simulink model "blance_leg2_machined"  (R2023a)
settings: Solver=VariableStepAuto  StartTime=0.0  StopTime=10  MaxStep=0.0050000000000000001  RelTol=5.0000000000000002e-05  AbsTol=9.9999999999999995e-07
InitFcn:
  | addpath(fileparts(get_param(bdroot,'FileName')));
  | apply_config(bdroot);
model workspace (MAT data in the model file):
  L_length_ref = timeseries
  L_length_ref.Name = 'unnamed'
  L_length_ref.DataInfo = tsdata.datametadata
  L_length_ref.DataInfo.Interpolation = tsdata.interpolation
  L_length_ref.DataInfo.Interpolation.Fhandle : function handle (value not decoded)
  L_length_ref.DataInfo.Interpolation.Name = 'linear'
  L_length_ref.TimeInfo = tsdata.timemetadata
  L_length_ref.TimeInfo.Length = 2
  L_length_ref.TimeInfo.DuplicateTimes = 0
  L_length_ref.TimeInfo.Time_ = [0; 10]
  L_length_ref.TimeInfo.Initialized = 1
  L_length_ref.QualityInfo = tsdata.qualmetadata
  L_length_ref.Data_ = [0.08; 0.08]
  L_v_ref = timeseries
  L_v_ref.Name = 'unnamed'
  L_v_ref.DataInfo = tsdata.datametadata
  L_v_ref.DataInfo.Interpolation = tsdata.interpolation
  L_v_ref.DataInfo.Interpolation.Fhandle : function handle (value not decoded)
  L_v_ref.DataInfo.Interpolation.Name = 'linear'
  L_v_ref.TimeInfo = tsdata.timemetadata
  L_v_ref.TimeInfo.Length = 3
  L_v_ref.TimeInfo.DuplicateTimes = 0
  L_v_ref.TimeInfo.Time_ = [0; 2; 5]
  L_v_ref.TimeInfo.Initialized = 1
  L_v_ref.QualityInfo = tsdata.qualmetadata
  L_v_ref.Data_ = [0; 2; 0]
  R_length_ref = timeseries
  R_length_ref.Name = 'unnamed'
  R_length_ref.DataInfo = tsdata.datametadata
  R_length_ref.DataInfo.Interpolation = tsdata.interpolation
  R_length_ref.DataInfo.Interpolation.Fhandle : function handle (value not decoded)
  R_length_ref.DataInfo.Interpolation.Name = 'linear'
  R_length_ref.TimeInfo = tsdata.timemetadata
  R_length_ref.TimeInfo.Length = 2
  R_length_ref.TimeInfo.DuplicateTimes = 0
  R_length_ref.TimeInfo.Time_ = [0; 10]
  R_length_ref.TimeInfo.Initialized = 1
  R_length_ref.QualityInfo = tsdata.qualmetadata
  R_length_ref.Data_ = [0.08; 0.08]
  R_v_ref = timeseries
  R_v_ref.Name = 'unnamed'
  R_v_ref.DataInfo = tsdata.datametadata
  R_v_ref.DataInfo.Interpolation = tsdata.interpolation
  R_v_ref.DataInfo.Interpolation.Fhandle : function handle (value not decoded)
  R_v_ref.DataInfo.Interpolation.Name = 'linear'
  R_v_ref.TimeInfo = tsdata.timemetadata
  R_v_ref.TimeInfo.Length = 3
  R_v_ref.TimeInfo.DuplicateTimes = 0
  R_v_ref.TimeInfo.Time_ = [0; 2; 5]
  R_v_ref.TimeInfo.Initialized = 1
  R_v_ref.QualityInfo = tsdata.qualmetadata
  R_v_ref.Data_ = [0; 2; 0]
  runScenario_cfg_override = []
  wheel_speed_compensation = 1
values from neighbouring files (symbols this model uses):
  K = cachedK    [configured_lqr_gain.m]    (also in get_k_length.m = lqr(A,B,Q,R); matlab.mat = [-1.73670717704  -0.157075032659  -0.691811333866  -0.787613)
  N = NM + mp*diff(x + L*sin(theta),t,2)    [get_k_length.m]
  s = sin(phi3 - phi2)    [five_bar_geometry_rm.m]
undefined symbols (not defined in the file or in its folder): X, Y, Z
libraries: sm_lib x82, nesl_utility x35, slpidlib x2
(part 1 of 3)
settings Model: Creator=Hhop  LastModifiedBy=2024r9000p
settings SolverCC: AlgebraicLoopSolver=TrustRegion  MinimalZcImpactIntegration=on
settings DebuggingCC: ReadBeforeWriteMsg=DisableAll  WriteAfterWriteMsg=DisableAll  WriteAfterReadMsg=DisableAll  MultiTaskDSMMsg=none
settings ModelReferenceCC: UpdateModelReferenceTargets=IfOutOfDate
settings SFSimCC: SFSimEcho=off
settings RTWCC: DLArmComputeVersion=19.05
settings ExplorerConfigSet: InternalSimMechanicsExplorerSettings="<ExplorerConfiguration><canonicalview>default</canonicalview><AnimationSetting><BasePlaybackSpeed>1.0</BasePlaybackSpeed><PlaybackSpeedFactor>1.0</PlaybackSpeedFactor></AnimationSetting><TilePanel><TileInfo><Tiles Columns=\"1\" Count=\"1\" Rows=\"1\"><Column Weight=\"1\"/><Row Weight=\"1\"/><Tile Height=\"1\" Width=\"1\" X=\"0\" Y=\"0\"/></Tiles></TileInfo><SceneInfo><SceneViewer><BGColor><R>0.60000002384185791</R><G>0.60000002384185791</G><B>0.60000002384185791</B></BGColor><Camera><DoPerspective>on</DoPerspective><Position><X>0.799859824006459164</X><Y>3.18443911570358829</Y><Z>0.15361581150017517</Z></Position><Center><X>-0.000140175993540658794</X><Y>3.18443911570358829</Y><Z>0.15361581150017517</Z></Center><Up><X>0</X><Y>0</Y><Z>1</Z></Up><ViewLimDist>1</ViewLimDist><YLim>0.466307658154998583</YLim><XLim>0.83228851713119445</XLim></Camera></SceneViewer></SceneInfo></TilePanel><MechEditorPanel><Cameras><Camera><Id>Camera1</Id><Value><Name>Camera1</Name><NativeCamera><PositionTrackingFeature>blance_leg_model.Rigid_Transform6.F</PositionTrackingFeature><CenterTrackingFeature>blance_leg_model.pitch.B</CenterTrackingFeature><UpVectorTrackingFeature>blance_leg_model.World_Frame1.W</UpVectorTrackingFeature><CenterTrackingOrigin>on</CenterTrackingOrigin><UpVectorTrackingDirection>+Z</UpVectorTrackingDirection></NativeCamera></Value></Camera></Cameras><GfxPanelCameraMap><MapElement CameraMLId=\"Camera1\" GfxPanelIndex=\"0\"/></GfxPanelCameraMap><VideoCreator><PlaybackSpeedRatio>1.0</PlaybackSpeedRatio><FrameRate>30</FrameRate><VideoFormat>Motion JPEG AVI</VideoFormat><FrameSize>auto</FrameSize></VideoCreator></MechEditorPanel></ExplorerConfiguration>"

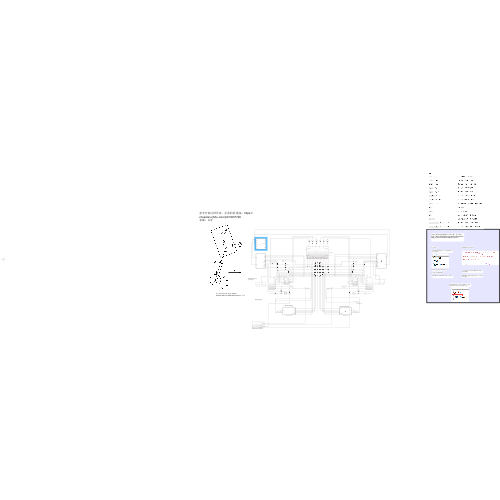
[thumbnail: Simulink's stored preview of the top-level diagram]
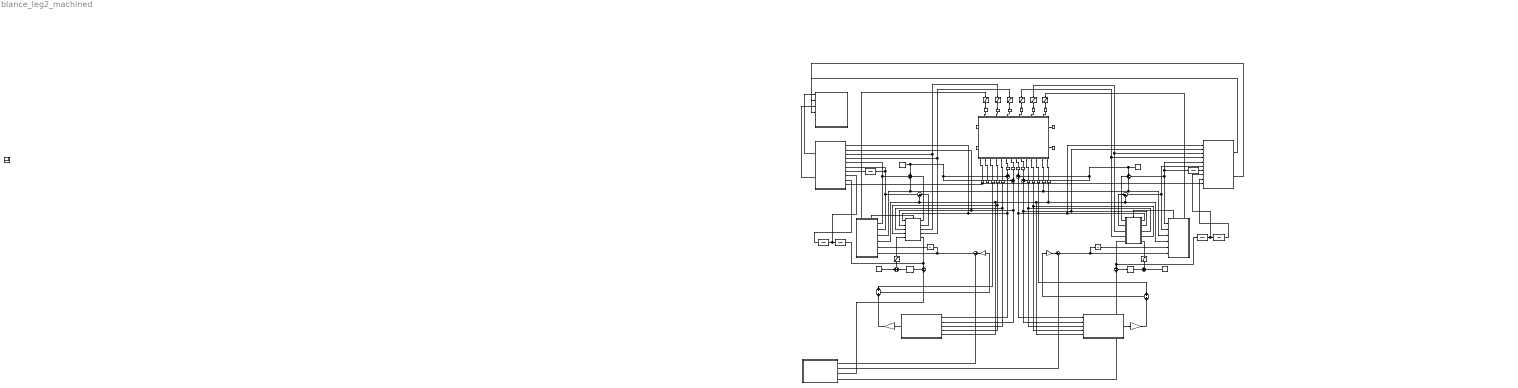
== system blance_leg2_machined ==
  note: 左侧支架对地角速度
  note: 状态目标设置
  note: 二阶系统
  note: LQR输出驱动轮转矩
      | 与虚拟杠转矩
  note: 参考开源文档作者：韭菜的菜 链接：https://zhuanlan.zhihu.com/p/613007726 来源：知乎
  note: 图片来源韭菜的菜 链接：https://zhuanlan.zhihu.com/p/613007726来源：知乎
  note: 运行步骤 :
  note: 所有开源文件必须置于同一文件夹(最好不要使用中文路径)
  note: 得到K参数后进入simulink 点击“运行”开始仿真
  note: addpath'(你所要想添加到的路径)'，具体用法可自行搜索
  note: 如果遇到如下图所示错误
  note: 可点击将其文件夹添加到MATLAB，或输入代码更换路径
  note: K = get_k_length(0.08)
  note: 在命令行窗口运行下图所示代码
  note: 如果想获取K矩阵关于腿长的函数的三次多项式系数在命令行窗口运行下图所示文件
  note: 该仿真是在b站轮腿机器人仿真开源上进行修改，链接：https://www.bilibili.com/read/cv26677904/?spm_id_from=333.999.0.0&jump_opus=1
  note: 右侧支架对地角速度
  Constant10 : Constant  Value=pi/2
  Constant12 : Constant  Value=pi/2
  Gain : Gain  Gain=-0.0603
  Gain1 : Gain  Gain=-0.0603
  Integrator1 : Integrator
  Integrator3 : Integrator
  Left Carrier Compensation Enable : Gain  Gain=wheel_speed_compensation
  Left Ground Wheel Omega : Sum
  Left Wheel Carrier Rate : MATLAB Function  TreatAsAtomicUnit=on
  MATLAB Function : MATLAB Function  TreatAsAtomicUnit=on
  MATLAB Function1 : MATLAB Function  TreatAsAtomicUnit=on
  MATLAB Function2 : MATLAB Function  TreatAsAtomicUnit=on
  PID Controller2 : slpidlib/PID Controller  Controller=PID  Form=Parallel  TimeDomain=Continuous-time  UseExternalTs=off  SampleTime=-1  IntegratorMethod=Forward Euler  FilterMethod=Forward Euler  ControllerParametersSource=internal  P=220  I=0  UseKiTs=off  D=1000  N=100  UseFilter=on  TunerSelectOption=Transfer Function Based (PID Tuner App)  InitialConditionSource=internal  InitialConditionForIntegrator=0  InitialConditionForFilter=0  DifferentiatorICPrevScaledInput=0  ExternalReset=none  TrackingMode=off  Kt=1  LimitOutput=off  SatLimitsSource=internal  UpperSaturationLimit=inf  LowerSaturationLimit=-inf  LinearizeAsGain=on  AntiWindupMode=none  Kb=1  LimitIntegrator=off  UpperIntegratorSaturationLimit=inf  LowerIntegratorSaturationLimit=-inf  POutMin=[]  POutMax=[]  IOutMin=[]  IOutMax=[]  DOutMin=[]  DOutMax=[]  NOutMin=[]  NOutMax=[]  SumOutMin=[]  SumOutMax=[]  SaturationOutMin=[]  SaturationOutMax=[]  PParamMin=[]  PParamMax=[]  IParamMin=[]  IParamMax=[]  DParamMin=[]  DParamMax=[]  NParamMin=[]  NParamMax=[]  KbParamMin=[]  KbParamMax=[]  KtParamMin=[]  KtParamMax=[]  KbOutMin=[]  KbOutMax=[]  KtOutMin=[]  KtOutMax=[]  IntegratorOutMin=[]  IntegratorOutMax=[]  FilterOutMin=[]  FilterOutMax=[]  SumI1OutMin=[]  SumI1OutMax=[]  SumI2OutMin=[]  SumI2OutMax=[]  SumI3OutMin=[]  SumI3OutMax=[]  SumI4OutMin=[]  SumI4OutMax=[]  SumDOutMin=[]  SumDOutMax=[]  DifferentiatorOutMin=[]  DifferentiatorOutMax=[]  FilterDiffOutCoefMin=[]  FilterDiffOutCoefMax=[]  ReciprocalOutMin=[]  ReciprocalOutMax=[]  SumDenOutMin=[]  SumDenOutMax=[]  SumNumOutMin=[]  SumNumOutMax=[]  DivideOutMin=[]  DivideOutMax=[]  UdiffTsProdOutMin=[]  UdiffTsProdOutMax=[]  NTsProdOutMin=[]  NTsProdOutMax=[]  UintegralTsProdOutMin=[]  UintegralTsProdOutMax=[]  UngainTsProdOutMin=[]  UngainTsProdOutMax=[]  ClampingZeroOutDataTypeStr=Inherit: Inherit via back propagation  ClampingZeroOutMin=[]  ClampingZeroOutMax=[]  FilterDenConstantOutDataTypeStr=Inherit: Inherit via back propagation  FilterDenConstantOutMin=[]  FilterDenConstantOutMax=[]  PCopyOutDataTypeStr=Inherit: Inherit via back propagation  PCopyOutMin=[]  PCopyOutMax=[]  NCopyOutDataTypeStr=Inherit: Inherit via back propagation  NCopyOutMin=[]  NCopyOutMax=[]  IntegratorContinuousStateAttributes=''  IntegratorStateMustResolveToSignalObject=off  IntegratorRTWStateStorageClass=Auto  FilterContinuousStateAttributes=''  FilterStateMustResolveToSignalObject=off  FilterRTWStateStorageClass=Auto  ParallelPVariant=InternalParameters  IdealPVariant=Disabled  IVariant=InternalParameters  DVariant=InternalParameters  IntegratorVariant=Continuous  SatVariant=Disabled  AWVariant=Passthrough  PCopyVariant=Disabled  TRVariant=Disabled  FdbkBlocksVariant=Forward  IdealPFdbkVariant=Disabled  SatFdbkVariant=Disabled  DerivativeFilterVariant=ContFilter  NVariant=InternalParameters  NCopyVariant=Disabled  FilterICVariant=InternalICsFilter  IntegratorICVariant=InternalICs  ExternalResetVariant=Disabled  TRSumVariant=Passthrough  SumFdbkVariant=Disabled  SumVariant=Sum_PID  TsampFilterVariant=InternalTs  TsampNgainVariant=Passthrough  TsampIntegralVariant=Disabled_SignalSpec  ExternalSaturationOutDataTypeStr=Inherit: Same as second input
  PID Controller3 : slpidlib/PID Controller  Controller=PID  Form=Parallel  TimeDomain=Continuous-time  UseExternalTs=off  SampleTime=-1  IntegratorMethod=Forward Euler  FilterMethod=Forward Euler  ControllerParametersSource=internal  P=220  I=0  UseKiTs=off  D=1000  N=100  UseFilter=on  TunerSelectOption=Transfer Function Based (PID Tuner App)  InitialConditionSource=internal  InitialConditionForIntegrator=0  InitialConditionForFilter=0  DifferentiatorICPrevScaledInput=0  ExternalReset=none  TrackingMode=off  Kt=1  LimitOutput=off  SatLimitsSource=internal  UpperSaturationLimit=inf  LowerSaturationLimit=-inf  LinearizeAsGain=on  AntiWindupMode=none  Kb=1  LimitIntegrator=off  UpperIntegratorSaturationLimit=inf  LowerIntegratorSaturationLimit=-inf  POutMin=[]  POutMax=[]  IOutMin=[]  IOutMax=[]  DOutMin=[]  DOutMax=[]  NOutMin=[]  NOutMax=[]  SumOutMin=[]  SumOutMax=[]  SaturationOutMin=[]  SaturationOutMax=[]  PParamMin=[]  PParamMax=[]  IParamMin=[]  IParamMax=[]  DParamMin=[]  DParamMax=[]  NParamMin=[]  NParamMax=[]  KbParamMin=[]  KbParamMax=[]  KtParamMin=[]  KtParamMax=[]  KbOutMin=[]  KbOutMax=[]  KtOutMin=[]  KtOutMax=[]  IntegratorOutMin=[]  IntegratorOutMax=[]  FilterOutMin=[]  FilterOutMax=[]  SumI1OutMin=[]  SumI1OutMax=[]  SumI2OutMin=[]  SumI2OutMax=[]  SumI3OutMin=[]  SumI3OutMax=[]  SumI4OutMin=[]  SumI4OutMax=[]  SumDOutMin=[]  SumDOutMax=[]  DifferentiatorOutMin=[]  DifferentiatorOutMax=[]  FilterDiffOutCoefMin=[]  FilterDiffOutCoefMax=[]  ReciprocalOutMin=[]  ReciprocalOutMax=[]  SumDenOutMin=[]  SumDenOutMax=[]  SumNumOutMin=[]  SumNumOutMax=[]  DivideOutMin=[]  DivideOutMax=[]  UdiffTsProdOutMin=[]  UdiffTsProdOutMax=[]  NTsProdOutMin=[]  NTsProdOutMax=[]  UintegralTsProdOutMin=[]  UintegralTsProdOutMax=[]  UngainTsProdOutMin=[]  UngainTsProdOutMax=[]  ClampingZeroOutDataTypeStr=Inherit: Inherit via back propagation  ClampingZeroOutMin=[]  ClampingZeroOutMax=[]  FilterDenConstantOutDataTypeStr=Inherit: Inherit via back propagation  FilterDenConstantOutMin=[]  FilterDenConstantOutMax=[]  PCopyOutDataTypeStr=Inherit: Inherit via back propagation  PCopyOutMin=[]  PCopyOutMax=[]  NCopyOutDataTypeStr=Inherit: Inherit via back propagation  NCopyOutMin=[]  NCopyOutMax=[]  IntegratorContinuousStateAttributes=''  IntegratorStateMustResolveToSignalObject=off  IntegratorRTWStateStorageClass=Auto  FilterContinuousStateAttributes=''  FilterStateMustResolveToSignalObject=off  FilterRTWStateStorageClass=Auto  ParallelPVariant=InternalParameters  IdealPVariant=Disabled  IVariant=InternalParameters  DVariant=InternalParameters  IntegratorVariant=Continuous  SatVariant=Disabled  AWVariant=Passthrough  PCopyVariant=Disabled  TRVariant=Disabled  FdbkBlocksVariant=Forward  IdealPFdbkVariant=Disabled  SatFdbkVariant=Disabled  DerivativeFilterVariant=ContFilter  NVariant=InternalParameters  NCopyVariant=Disabled  FilterICVariant=InternalICsFilter  IntegratorICVariant=InternalICs  ExternalResetVariant=Disabled  TRSumVariant=Passthrough  SumFdbkVariant=Disabled  SumVariant=Sum_PID  TsampFilterVariant=InternalTs  TsampNgainVariant=Passthrough  TsampIntegralVariant=Disabled_SignalSpec  ExternalSaturationOutDataTypeStr=Inherit: Same as second input
  PS-Simulink Converter{1,18,20..22,24,27..37} (17 alike) : nesl_utility/PS-Simulink Converter  PhysicalDomain=network_engine_domain  SubClassName=ps_output  LeftPortType=input  RightPortType=output  PseudoPeriodic=off  Frequencies=[]  VectorFormat=1-D array  Unit=inherit  AffineConversion=off
  PS-Simulink Converter19 : nesl_utility/PS-Simulink Converter  Tag=1  PhysicalDomain=network_engine_domain  SubClassName=ps_output  LeftPortType=input  RightPortType=output  PseudoPeriodic=off  Frequencies=[]  VectorFormat=1-D array  Unit=inherit  AffineConversion=off
  Right Carrier Compensation Enable : Gain  Gain=wheel_speed_compensation
  Right Ground Wheel Omega : Sum
  Right Wheel Carrier Rate : MATLAB Function  TreatAsAtomicUnit=on
  Saturation{1..4} (4 alike) : Saturate  UpperLimit=100  LowerLimit=-100
  Saturation5 : Saturate  UpperLimit=300  LowerLimit=-300
  Saturation6 : Saturate  UpperLimit=300  LowerLimit=-300
  Saturation7 : Saturate  UpperLimit=9  LowerLimit=-9
  Saturation8 : Saturate  UpperLimit=9  LowerLimit=-9
  Scenario References : Subsystem
  Simulink-PS Converter{1..6} (6 alike) : nesl_utility/Simulink-PS Converter  PhysicalDomain=network_engine_domain  SubClassName=ps_input  LeftPortType=input  RightPortType=output  PseudoPeriodic=off  Frequencies=[]  NoiseDistribution=none  NoiseParameters=[]  Unit=1  AffineConversion=off  FilteringAndDerivatives=provide  SimscapeFilterOrder=1  InputFilterTimeConstant=0.001  UdotUserProvided=0
  Subsystem1 : Subsystem
      settings: PortSchema="{\"entries\":[{\"content\":{\"sides\":[{\"content\":{\"connectorIds\":[\"In1\",\"In2\",\"In3\",\"In4\",\"In5\",\"In6\"]},\"type\":\"ConnectorPlacement.EquallySpacedRectSide\",\"uuid\":\"055cb80c-cd03-4a8d-aef8-6b3df8c72d3f\"},{\"content\":{\"connectorIds\":[],\"side\":\"RIGHT\"},\"type\":\"ConnectorPlacement.EquallySpacedRectSide\",\"uuid\":\"5756fad1-d70f-4a11-a5af-d2f67bfb0d7e\"},{\"content\":{\"connectorIds\":[\"Out1\",\"Out2\"],\"side\":\"TOP\"},\"type\":\"ConnectorPlacement.EquallySpacedRectSide\",\"uuid\":\"9c70cf42-10f8-4525-9406-562484abf580\"}]},\"type\":\"ConnectorPlacement.EquallySpacedConnector\",\"uuid\":\"7084d402-0e44-4d2f-8cc2-1336d196e84d\"}],\"packageUris\":[\"http://schema.mathworks.com/mf0/Connector/R2020b\"],\"version\":\"1.0\"}"
  Subsystem4 : Subsystem
      settings: PortSchema="{\"entries\":[{\"content\":{\"sides\":[{\"content\":{\"connectorIds\":[\"In1\",\"In2\",\"In3\",\"In4\",\"In5\"]},\"type\":\"ConnectorPlacement.EquallySpacedRectSide\",\"uuid\":\"40de31e0-cc19-460f-99e9-affbb47f7204\"},{\"content\":{\"connectorIds\":[\"Out1\",\"Out2\",\"Out3\",\"Out4\",\"Out5\"],\"side\":\"RIGHT\"},\"type\":\"ConnectorPlacement.EquallySpacedRectSide\",\"uuid\":\"e61df4ab-633d-456a-aa2d-223df880274d\"},{\"content\":{\"connectorIds\":[\"In6\"],\"side\":\"TOP\"},\"type\":\"ConnectorPlacement.EquallySpacedRectSide\",\"uuid\":\"a7334146-3144-4ab1-9f08-8bf1583597b4\"}]},\"type\":\"ConnectorPlacement.EquallySpacedConnector\",\"uuid\":\"1490fe93-b025-4c86-96e6-b1bfc13c7f50\"}],\"packageUris\":[\"http://schema.mathworks.com/mf0/Connector/R2020b\"],\"version\":\"1.0\"}"
  Sum1 : Sum  Inputs=|+-
  Sum13 : Sum  Inputs=++|
  Sum14 : Sum  Inputs=|++
  Sum15 : Sum  Inputs=|++
  Sum16 : Sum  Inputs=|--
  Sum17 : Sum  Inputs=+--
  Sum18 : Sum  Inputs=+|+
  Sum2 : Sum  Inputs=|+-
  Sum20 : Sum  Inputs=++|
  Sum23 : Sum  Inputs=-|+
  Sum24 : Sum  Inputs=+--
  Sum25 : Sum  Inputs=+|+
  Sum27 : Sum  Inputs=|--
  Sum29 : Sum  Inputs=-|+
  Transfer Fcn{,1..5} (6 alike) : TransferFcn  Denominator=[1 1]
  blance_leg_model : Subsystem
      settings: PortSchema="{\"entries\":[{\"content\":{\"sides\":[{\"content\":{\"connectorIds\":[\"LConn1\",\"LConn2\",\"LConn3\",\"LConn4\",\"LConn5\",\"LConn6\"]},\"type\":\"ConnectorPlacement.EquallySpacedRectSide\",\"uuid\":\"df2d0b15-ec70-4430-8d90-67c6d88950b4\"},{\"content\":{\"connectorIds\":[\"RConn1\",\"RConn2\",\"RConn3\",\"RConn4\",\"RConn5\",\"RConn6\",\"RConn7\",\"RConn8\",\"RConn9\",\"RConn10\",\"RConn11\",\"RConn12\",\"RConn13\",\"RConn14\"],\"side\":\"RIGHT\"},\"type\":\"ConnectorPlacement.EquallySpacedRectSide\",\"uuid\":\"ec9b4787-d265-4ad9-b676-e253d2304993\"},{\"content\":{\"connectorIds\":[\"LConn7\",\"LConn8\"],\"side\":\"TOP\"},\"type\":\"ConnectorPlacement.EquallySpacedRectSide\",\"uuid\":\"40dd08fe-dc32-4cee-bbb8-c1ec6d04ee32\"},{\"content\":{\"connectorIds\":[\"RConn15\",\"RConn16\"],\"side\":\"BOTTOM\"},\"type\":\"ConnectorPlacement.EquallySpacedRectSide\",\"uuid\":\"0f9c1faf-3e52-4dca-bbb1-0993be9fa88c\"}]},\"type\":\"ConnectorPlacement.EquallySpacedConnector\",\"uuid\":\"d540d646-85aa-4f97-ae4d-1bccec971368\"}],\"packageUris\":[\"http://schema.mathworks.com/mf0/Connector/R2020b\"],\"version\":\"1.0\"}"
  calc : Subsystem
      settings: PortSchema="{\"entries\":[{\"content\":{\"sides\":[{\"content\":{\"connectorIds\":[\"In1\",\"In2\",\"In3\",\"In4\",\"In5\",\"In6\"]},\"type\":\"ConnectorPlacement.EquallySpacedRectSide\",\"uuid\":\"055cb80c-cd03-4a8d-aef8-6b3df8c72d3f\"},{\"content\":{\"connectorIds\":[],\"side\":\"RIGHT\"},\"type\":\"ConnectorPlacement.EquallySpacedRectSide\",\"uuid\":\"5756fad1-d70f-4a11-a5af-d2f67bfb0d7e\"},{\"content\":{\"connectorIds\":[\"Out1\",\"Out2\"],\"side\":\"TOP\"},\"type\":\"ConnectorPlacement.EquallySpacedRectSide\",\"uuid\":\"9c70cf42-10f8-4525-9406-562484abf580\"}]},\"type\":\"ConnectorPlacement.EquallySpacedConnector\",\"uuid\":\"7084d402-0e44-4d2f-8cc2-1336d196e84d\"}],\"packageUris\":[\"http://schema.mathworks.com/mf0/Connector/R2020b\"],\"version\":\"1.0\"}"
  control : Subsystem
      settings: PortSchema="{\"entries\":[{\"content\":{\"sides\":[{\"content\":{\"connectorIds\":[\"In1\",\"In2\",\"In3\",\"In4\",\"In5\"]},\"type\":\"ConnectorPlacement.EquallySpacedRectSide\",\"uuid\":\"40de31e0-cc19-460f-99e9-affbb47f7204\"},{\"content\":{\"connectorIds\":[\"Out1\",\"Out2\",\"Out3\",\"Out4\",\"Out5\"],\"side\":\"RIGHT\"},\"type\":\"ConnectorPlacement.EquallySpacedRectSide\",\"uuid\":\"e61df4ab-633d-456a-aa2d-223df880274d\"},{\"content\":{\"connectorIds\":[\"In6\"],\"side\":\"TOP\"},\"type\":\"ConnectorPlacement.EquallySpacedRectSide\",\"uuid\":\"a7334146-3144-4ab1-9f08-8bf1583597b4\"}]},\"type\":\"ConnectorPlacement.EquallySpacedConnector\",\"uuid\":\"1490fe93-b025-4c86-96e6-b1bfc13c7f50\"}],\"packageUris\":[\"http://schema.mathworks.com/mf0/Connector/R2020b\"],\"version\":\"1.0\"}"
  mean_x2 : Scope
  除去轮子后机体重量 : Constant  Value=9
  除去轮子后机体重量， : Constant  Value=9
  wires:
  除去轮子后机体重量，/1 -> Sum25/1
  Sum27/1 -> MATLAB Function1/6(d_theta), Subsystem1/2(d_theta)
  Constant12/1 -> Sum15/2, Sum14/2, Sum17/1
  Sum29/1 -> PID Controller3/1
  Sum16/1 -> calc/2(d_theta), MATLAB Function/6(d_theta), Transfer Fcn/1
  Sum24/1 -> MATLAB Function/5(theta), calc/1(theta)
  Constant10/1 -> Sum24/1, Sum20/1, Sum13/1
  Sum23/1 -> PID Controller2/1
  PID Controller2/1 -> Sum25/2
  Sum17/1 -> MATLAB Function1/5(theta), Transfer Fcn3/1, Subsystem1/1(theta)
  除去轮子后机体重量/1 -> Sum18/2
  PID Controller3/1 -> Sum18/1
  Saturation1/1 -> Simulink-PS Converter1/1
  Saturation2/1 -> Simulink-PS Converter3/1
  Saturation3/1 -> Simulink-PS Converter2/1
  Saturation4/1 -> Simulink-PS Converter5/1
  PS-Simulink Converter32/1 -> Sum13/2
  PS-Simulink Converter35/1 -> Sum15/1
  PS-Simulink Converter33/1 -> Sum14/1
  PS-Simulink Converter34/1 -> Sum20/2
  Sum13/1 -> Left Wheel Carrier Rate/1(phi1), MATLAB Function/1(phi1), control/1(phi1)  "左侧J1转角"
  Sum20/1 -> Left Wheel Carrier Rate/2(phi4), control/2(phi4), MATLAB Function/2(phi4)
  Sum14/1 -> Subsystem4/1(phi1), MATLAB Function1/1(phi1), Right Wheel Carrier Rate/1(phi1)
  Sum15/1 -> Subsystem4/2(phi4), MATLAB Function1/2(phi4), Right Wheel Carrier Rate/2(phi4)  "右侧髋关节1转角"
  PS-Simulink Converter31/1 -> Left Wheel Carrier Rate/3(w1), control/3(d_phi1)
  PS-Simulink Converter29/1 -> Left Wheel Carrier Rate/4(w4), control/4(d_phi4)
  PS-Simulink Converter20/1 -> Right Wheel Carrier Rate/3(w1), Subsystem4/3(d_phi1)
  PS-Simulink Converter21/1 -> Right Wheel Carrier Rate/4(w4), Subsystem4/4(d_phi4)
  PS-Simulink Converter28/1 -> Left Ground Wheel Omega/1  "左轮编码器相对角速度"
  PS-Simulink Converter22/1 -> Right Ground Wheel Omega/1  "右轮编码器相对角速度"
  PS-Simulink Converter1/1 -> Sum17/3, Subsystem1/3(phi), Sum24/3, calc/3(phi)
  PS-Simulink Converter24/1 -> Right Wheel Carrier Rate/5(bodyPitchRate), calc/4(d_phi), Sum16/2, Left Wheel Carrier Rate/5(bodyPitchRate), Subsystem1/4(d_phi), Sum27/2
  control/1(phi0) -> Sum24/2
  control/2(d_phi0) -> Sum16/1
  Subsystem4/1(phi0) -> Sum17/2
  Subsystem4/2(d_phi0) -> Sum27/1
  Subsystem4/5(L0) -> Transfer Fcn4/1, Sum29/1  "右轮腿长"
  calc/1(Tp) -> control/6(Tp)
  Sum18/1 -> Saturation5/1
  Sum25/1 -> Saturation6/1
  Saturation6/1 -> control/5(F0)
  control/3(T1) -> MATLAB Function/3(T1), Saturation1/1  "左侧髋关节1力矩"
  Subsystem4/3(T1) -> MATLAB Function1/3(T1), Saturation4/1  "右轮髋关节1力矩"
  control/4(T2) -> MATLAB Function/4(T2), Saturation2/1  "左侧髋关节2力矩"
  Subsystem4/4(T2) -> MATLAB Function1/4(T2), Saturation3/1  "右轮髋关节2力矩"
  calc/2(T) -> Saturation7/1
  Subsystem1/2(T) -> Saturation8/1
  Saturation7/1 -> Simulink-PS Converter6/1
  Saturation8/1 -> Simulink-PS Converter4/1
  Integrator3/1 -> calc/5(x)
  Gain1/1 -> Sum1/1  "左轮对地滚动速度估计"
  Sum1/1 -> calc/6(d_x), Integrator3/1  "左轮速度误差"
  Sum2/1 -> Integrator1/1, Subsystem1/6(d_x)  "右轮速度误差"
  Subsystem1/1(Tp) -> Subsystem4/6(Tp)
  Saturation5/1 -> Subsystem4/5(F0)
  Scenario References/3(L_length_ref) -> Sum23/2  "左轮目标腿长"
  Scenario References/4(R_length_ref) -> Sum29/2  "右轮目标腿长"
  Integrator1/1 -> Subsystem1/5(x)
  Scenario References/1(L_v_ref) -> Sum1/2  "左轮目标速度"
  Scenario References/2(R_v_ref) -> Sum2/2  "右轮目标速度"
  Left Wheel Carrier Rate/1(omega) -> Left Carrier Compensation Enable/1
  Left Carrier Compensation Enable/1 -> Left Ground Wheel Omega/2
  Right Wheel Carrier Rate/1(omega) -> Right Carrier Compensation Enable/1
  Right Carrier Compensation Enable/1 -> Right Ground Wheel Omega/2
  Right Ground Wheel Omega/1 -> Gain/1  "右轮补偿后对地角速度"
  control/5(L0) -> Transfer Fcn1/1, Sum23/1  "左轮腿长"
  Left Ground Wheel Omega/1 -> Gain1/1  "左轮补偿后对地角速度"
  Gain/1 -> Sum2/1  "右轮对地滚动速度估计"
  PS-Simulink Converter18/1 -> MATLAB Function/10(Z_M_Ddot), MATLAB Function1/10(Z_M_Ddot)
  Transfer Fcn/1 -> MATLAB Function/7(dd_theta)
  Transfer Fcn1/1 -> MATLAB Function/8(d_L0), Transfer Fcn2/1
  Transfer Fcn2/1 -> MATLAB Function/9(dd_L0)
  Transfer Fcn3/1 -> MATLAB Function1/7(dd_theta)
  Transfer Fcn4/1 -> MATLAB Function1/8(d_L0), Transfer Fcn5/1
  Transfer Fcn5/1 -> MATLAB Function1/9(dd_L0)
  MATLAB Function/1(F_N) -> MATLAB Function2/1(F_N_L)
  MATLAB Function1/1(F_N) -> MATLAB Function2/2(F_N_R)
  MATLAB Function/2(valid) -> MATLAB Function2/3(valid_L)
  MATLAB Function1/2(valid) -> MATLAB Function2/4(valid_R)
  connections:
  blance_leg_model/LConn2 -- Simulink-PS Converter1/RConn1
  blance_leg_model/LConn3 -- Simulink-PS Converter3/RConn1
  blance_leg_model/LConn4 -- Simulink-PS Converter2/RConn1
  blance_leg_model/LConn5 -- Simulink-PS Converter5/RConn1
  blance_leg_model/RConn10 -- PS-Simulink Converter20/LConn1
  blance_leg_model/RConn11 -- PS-Simulink Converter21/LConn1
  blance_leg_model/RConn2 -- PS-Simulink Converter19/LConn1
  blance_leg_model/RConn12 -- PS-Simulink Converter22/LConn1
  blance_leg_model/RConn3 -- PS-Simulink Converter28/LConn1
  blance_leg_model/RConn14 -- PS-Simulink Converter24/LConn1
  blance_leg_model/RConn5 -- PS-Simulink Converter31/LConn1
  blance_leg_model/RConn1 -- PS-Simulink Converter18/LConn1
  blance_leg_model/RConn4 -- PS-Simulink Converter29/LConn1
  blance_leg_model/RConn13 -- PS-Simulink Converter1/LConn1
  blance_leg_model/RConn6 -- PS-Simulink Converter32/LConn1
  blance_leg_model/RConn7 -- PS-Simulink Converter34/LConn1
  blance_leg_model/RConn8 -- PS-Simulink Converter33/LConn1
  blance_leg_model/RConn9 -- PS-Simulink Converter35/LConn1
  blance_leg_model/LConn7 -- PS-Simulink Converter27/LConn1
  blance_leg_model/LConn8 -- PS-Simulink Converter30/LConn1
  blance_leg_model/RConn15 -- PS-Simulink Converter36/LConn1
  blance_leg_model/RConn16 -- PS-Simulink Converter37/LConn1
  blance_leg_model/LConn1 -- Simulink-PS Converter6/RConn1
  blance_leg_model/LConn6 -- Simulink-PS Converter4/RConn1

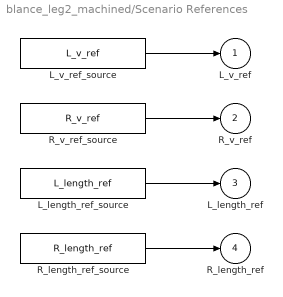
== system blance_leg2_machined/Scenario References ==
  L_length_ref_source : FromWorkspace  VariableName=L_length_ref  Interpolate=off  OutputAfterFinalValue=Holding final value
  L_v_ref_source : FromWorkspace  VariableName=L_v_ref  Interpolate=off  OutputAfterFinalValue=Holding final value
  R_length_ref_source : FromWorkspace  VariableName=R_length_ref  Interpolate=off  OutputAfterFinalValue=Holding final value
  R_v_ref_source : FromWorkspace  VariableName=R_v_ref  Interpolate=off  OutputAfterFinalValue=Holding final value
  L_v_ref : Outport
  R_v_ref : Outport  Port=2
  L_length_ref : Outport  Port=3
  R_length_ref : Outport  Port=4
  wires:
  L_v_ref_source/1 -> L_v_ref/1
  R_v_ref_source/1 -> R_v_ref/1
  L_length_ref_source/1 -> L_length_ref/1
  R_length_ref_source/1 -> R_length_ref/1

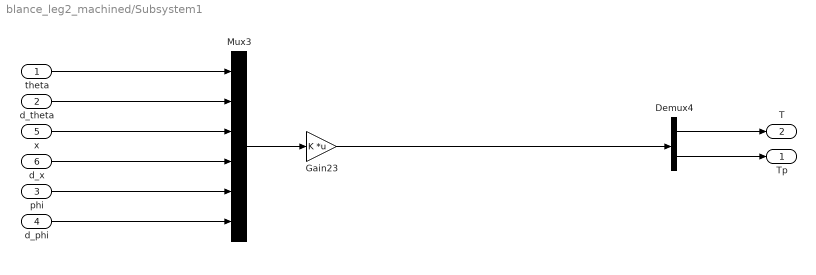
== system blance_leg2_machined/Subsystem1 ==
  theta : Inport
  d_theta : Inport  Port=2
  phi : Inport  Port=3
  d_phi : Inport  Port=4
  x : Inport  Port=5
  d_x : Inport  Port=6
  Demux4 : Demux  Outputs=2
  Gain23 : Gain  Gain=K  Multiplication=Matrix(K*u) (u vector)
  Mux3 : Mux  Inputs=6
  Tp : Outport
  T : Outport  Port=2
  wires:
  theta/1 -> Mux3/1
  d_theta/1 -> Mux3/2
  d_x/1 -> Mux3/4
  d_phi/1 -> Mux3/6
  phi/1 -> Mux3/5
  Demux4/2 -> Tp/1
  x/1 -> Mux3/3
  Mux3/1 -> Gain23/1
  Gain23/1 -> Demux4/1
  Demux4/1 -> T/1

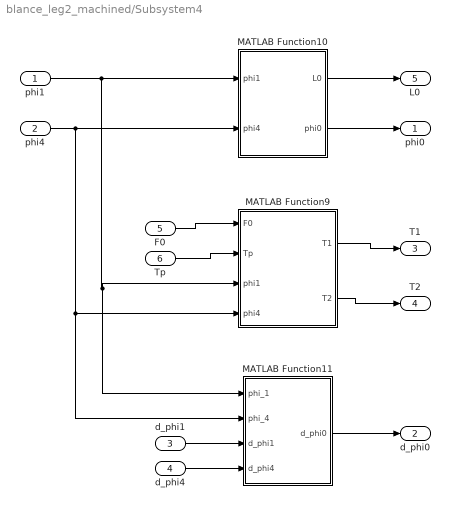
== system blance_leg2_machined/Subsystem4 ==
  phi1 : Inport
  phi4 : Inport  Port=2
  d_phi1 : Inport  Port=3
  d_phi4 : Inport  Port=4
  F0 : Inport  Port=5
  Tp : Inport  Port=6
  MATLAB Function10 : MATLAB Function  TreatAsAtomicUnit=on
  MATLAB Function11 : MATLAB Function  TreatAsAtomicUnit=on
  MATLAB Function9 : MATLAB Function  TreatAsAtomicUnit=on
  phi0 : Outport
  d_phi0 : Outport  Port=2
  T1 : Outport  Port=3
  T2 : Outport  Port=4
  L0 : Outport  Port=5
  wires:
  phi1/1 -> MATLAB Function11/1(phi_1), MATLAB Function9/3(phi1), MATLAB Function10/1(phi1)
  MATLAB Function10/2(phi0) -> phi0/1
  MATLAB Function11/1(d_phi0) -> d_phi0/1
  Tp/1 -> MATLAB Function9/2(Tp)
  d_phi4/1 -> MATLAB Function11/4(d_phi4)
  d_phi1/1 -> MATLAB Function11/3(d_phi1)
  MATLAB Function9/1(T1) -> T1/1
  phi4/1 -> MATLAB Function11/2(phi_4), MATLAB Function9/4(phi4), MATLAB Function10/2(phi4)
  F0/1 -> MATLAB Function9/1(F0)
  MATLAB Function9/2(T2) -> T2/1
  MATLAB Function10/1(L0) -> L0/1
